simulink subsystem "BatteryHV_SystemTable_refsub"  (R2025b)
settings: Solver=VariableStepAuto  StartTime=0.0  StopTime=10.0  RelTol=1e-3
undefined symbols (not defined in the file or in its folder): batteryHV, initial, Minus, Plus
libraries: fl_lib x24, nesl_utility x10, batteryecm_lib x1
settings Model: Creator=isaacito  LastModifiedBy=isaacito
settings OptimizationCC: ReuseModelBlockBuffer=off
settings RTWCC: GPUComputeCapability=3.5

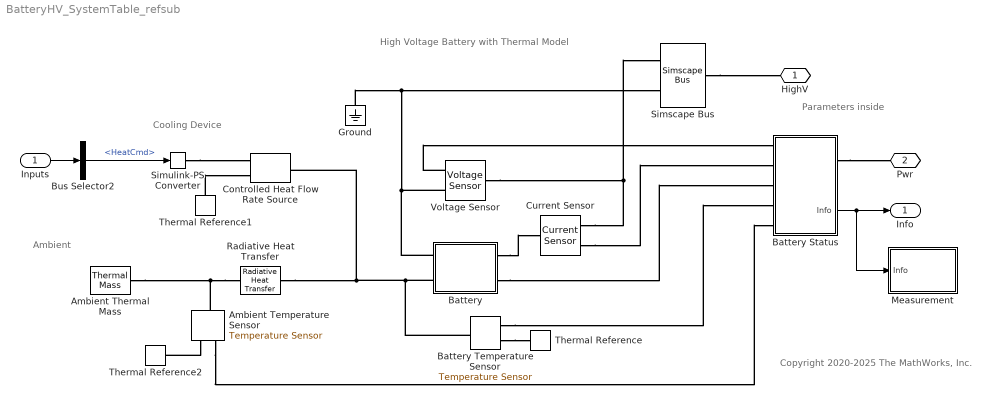
== system BatteryHV_SystemTable_refsub ==
  note: High Voltage Battery with Thermal Model
  note: Ambient
  note: Cooling Device
  note: Copyright 2020-2025 The MathWorks, Inc.
  note: Parameters inside
  Inputs : Inport
  Ambient Temperature Sensor : fl_lib/Thermal/Thermal Sensors/Temperature Sensor  temperature_measure=foundation.enum.MeasurementReference.difference
  Ambient Thermal Mass : fl_lib/Thermal/Thermal Elements/Thermal Mass  mass_type=foundation.enum.constant_variable.constant  mass=batteryHV.ambientMass_t t  sp_heat=batteryHV.ambientSpecificHeat_J_per_Kkg J/(K*kg)  mass_min=1e-6 kg  num_ports=foundation.enum.numPorts2.one  m_specify=off  m_priority=High  m=1 kg  m_nominal_specify=off  m_nominal_value=1  m_nominal_unit=kg  T_specify=on  T_priority=High  T=initial.ambientTemp_K K  T_nominal_specify=off  T_nominal_value=1  T_nominal_unit=K  Q_specify=off  Q_priority=None  Q=0 W  Q_nominal_specify=off  Q_nominal_value=1  Q_nominal_unit=W
  Battery : Subsystem
  Battery Status : Subsystem
      settings: PortSchema="{\"entries\":[{\"content\":{\"sides\":[{\"content\":{\"connectorIds\":[\"LConn1\",\"LConn2\",\"LConn3\",\"LConn4\",\"LConn5\"]},\"type\":\"ConnectorPlacement.EquallySpacedRectSide\",\"uuid\":\"ceb40bee-a67a-415b-b9a3-f68aa0f1718c\"},{\"content\":{\"connectorIds\":[\"RConn1\",\"Out1\"],\"side\":\"RIGHT\"},\"type\":\"ConnectorPlacement.EquallySpacedRectSide\",\"uuid\":\"395c2f85-e3a4-4d83-be11-c4910c287b37\"},{\"content\":{\"side\":\"TOP\"},\"type\":\"ConnectorPlacement.EquallySpacedRectSide\",\"uuid\":\"f70bb581-3c81-49dd-9a63-28b015635667\"}]},\"type\":\"ConnectorPlacement.EquallySpacedConnector\",\"uuid\":\"f11b0a3f-3785-405e-864d-e7b7ac2aade7\"}],\"packageUris\":[\"http://schema.mathworks.com/mf0/Connector/R2020b\"],\"version\":\"1.0\"}"
  Battery Temperature Sensor : fl_lib/Thermal/Thermal Sensors/Temperature Sensor  temperature_measure=foundation.enum.MeasurementReference.difference
  Bus Selector2 : BusSelector  OutputSignals=HeatCmd
  Controlled Heat Flow Rate Source : fl_lib/Thermal/Thermal Sources/Controlled Heat Flow Rate Source
  Current Sensor : fl_lib/Electrical/Electrical Sensors/Current Sensor
  Ground : fl_lib/Electrical/Electrical Elements/Electrical Reference
  Measurement : Subsystem
  Radiative Heat Transfer : fl_lib/Thermal/Thermal Elements/Radiative Heat Transfer  area=batteryHV.RadiationArea_m2 m^2  rad_tr_coeff=batteryHV.RadiationCoeff_W_per_K4m2 W/(K^4*m^2)  T_specify=off  T_priority=None  T=0 K  T_nominal_specify=off  T_nominal_value=1  T_nominal_unit=K  Q_specify=off  Q_priority=None  Q=0 W  Q_nominal_specify=off  Q_nominal_value=1  Q_nominal_unit=W
      settings: InternalSimscapePortConfiguration="{\"Bottom\":[],\"Left\":[{\"id\":\"A\",\"label\":\"A\",\"type\":\"foundation.thermal.thermal\"}],\"Right\":[{\"id\":\"B\",\"label\":\"B\",\"type\":\"foundation.thermal.thermal\"}],\"Top\":[]}"
  Simscape Bus : SimscapeBus  HierarchyStrings=Plus;Minus  ConnectionType=Bus: Bus_HighVoltage
      settings: AttributesFormatString=%<ConnectionType>
  Simulink-PS Converter : nesl_utility/Simulink-PS Converter  PhysicalDomain=network_engine_domain  SubClassName=ps_input  LeftPortType=input  RightPortType=output  PseudoPeriodic=off  Frequencies=[]  NoiseDistribution=none  NoiseParameters=[]  Unit=W  AffineConversion=off  FilteringAndDerivatives=provide  SimscapeFilterOrder=1  InputFilterTimeConstant=0.001  UdotUserProvided=0
  Thermal Reference : fl_lib/Thermal/Thermal Elements/Thermal Reference
  Thermal Reference1 : fl_lib/Thermal/Thermal Elements/Thermal Reference
  Thermal Reference2 : fl_lib/Thermal/Thermal Elements/Thermal Reference
  Voltage Sensor : fl_lib/Electrical/Electrical Sensors/Voltage Sensor
  HighV : PMIOPort  Side=Right
  Pwr : PMIOPort  Port=2  Side=Right
  Info : Outport
  wires:
  Bus Selector2/1 -> Simulink-PS Converter/1  "<HeatCmd>"
  Inputs/1 -> Bus Selector2/1
  Battery Status/1(Info) -> Info/1, Measurement/1(Info)
  connections:
  Ground/LConn1 -- Simscape Bus/LConn2 -- Voltage Sensor/RConn2 -- Battery/RConn1
  Voltage Sensor/LConn1 -- Simscape Bus/LConn1 -- Current Sensor/RConn2
  Battery Temperature Sensor/LConn1 -- Controlled Heat Flow Rate Source/LConn1 -- Radiative Heat Transfer/RConn1 -- Battery/RConn2
  Radiative Heat Transfer/LConn1 -- Ambient Thermal Mass/LConn1 -- Ambient Temperature Sensor/LConn1
  Simscape Bus/RConn1 -- HighV/RConn1
  Ambient Temperature Sensor/RConn1 -- Thermal Reference2/LConn1
  Simulink-PS Converter/RConn1 -- Controlled Heat Flow Rate Source/RConn1
  Thermal Reference1/LConn1 -- Controlled Heat Flow Rate Source/RConn2
  Voltage Sensor/RConn1 -- Battery Status/LConn1
  Current Sensor/RConn1 -- Battery Status/LConn2
  Battery Temperature Sensor/RConn1 -- Thermal Reference/LConn1
  Battery Temperature Sensor/RConn2 -- Battery Status/LConn4
  Ambient Temperature Sensor/RConn2 -- Battery Status/LConn5
  Battery/LConn2 -- Battery Status/LConn3
  Battery/LConn1 -- Current Sensor/LConn1
  Battery Status/RConn1 -- Pwr/RConn1

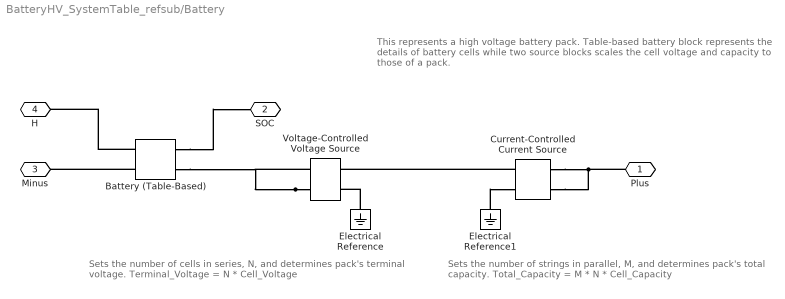
== system BatteryHV_SystemTable_refsub/Battery ==
  note: This represents a high voltage battery pack.
      | Table-based battery block represents the details of
      | battery cells while two source blocks scales
      | the cell voltage and capacity to those of a pack.
  note: Sets the number of strings in parallel, M,
      | and determines pack's total capacity.
      | Total_Capacity = M * N * Cell_Capacity
  note: Sets the number of cells in series, N,
      | and determines pack's terminal voltage.
      | Terminal_Voltage = N * Cell_Voltage
  Battery (Table-Based) : batteryecm_lib/Battery (Table-Based)  SOC_vec=batteryHV.SOC_normalized  T_dependence=simscape.enum.tablebattery.temperature_dependence.yes  prm_dir=simscape.enum.tablebattery.prm_dir.noCurrentDirectionality  T_vec=batteryHV.Temperatures_degC degC  V0_mat=batteryHV.OpenCircuitVoltage_V V  V0_vec=[3.5057, 3.566, 3.6337, 3.7127, 3.9259, 4.0777, 4.1928] V  V_range=[0, inf] V  R0_mat=batteryHV.TerminalResistance_Ohm Ohm  R0_vec=[.0085, .0085, .0087, .0082, .0083, .0085, .0085] Ohm  R0_dis_mat=[.0117, .0085, .009; .011, .0085, .009; .0114, .0087, .0092; .0107, .0082, .0088; .0107, .0083, .0091; .0113, .0085, .0089; .0116, .0085, .0089] Ohm  R0_dis_vec=[.0085, .0085, .0087, .0082, .0083, .0085, .0085] Ohm  R0_ch_mat=[.0117, .0085, .009; .011, .0085, .009; .0114, .0087, .0092; .0107, .0082, .0088; .0107, .0083, .0091; .0113, .0085, .0089; .0116, .0085, .0089] Ohm  R0_ch_vec=[.0085, .0085, .0087, .0082, .0083, .0085, .0085] Ohm  AH=batteryHV.CellCharge_Ahr A*hr  prm_leak=simscape.enum.tablebattery.prm_leak.disabled  Rleak_vec=[8000, 7000, 6000] Ohm  Rleak=7e3 Ohm  extrapolation_option=simscape.enum.extrapolation.nearest  SOC_port=simscape.enum.tablebattery.enable.yes  prm_dyn=simscape.enum.tablebattery.prm_dyn.off  R1_mat=[.0109, .0029, .0013; .0069, .0024, .0012; .0047, .0026, .0013; .0034, .0016, .001; .0033, .0023, .0014; .0033, .0018, .0011; .0028, .0017, .0011] Ohm  R1_vec=[.0029, .0024, .0026, .0016, .0023, .0018, .0017] Ohm  tau1_mat=[20, 36, 39; 31, 45, 39; 109, 105, 61; 36, 29, 26; 59, 77, 67; 40, 33, 29; 25, 39, 33] s  tau1_vec=[36, 45, 105, 29, 77, 33, 39] s  R2_mat=[.0109, .0029, .0013; .0069, .0024, .0012; .0047, .0026, .0013; .0034, .0016, .001; .0033, .0023, .0014; .0033, .0018, .0011; .0028, .0017, .0011] Ohm  R2_vec=[.0029, .0024, .0026, .0016, .0023, .0018, .0017] Ohm  tau2_mat=[20, 36, 39; 31, 45, 39; 109, 105, 61; 36, 29, 26; 59, 77, 67; 40, 33, 29; 25, 39, 33] s  tau2_vec=[36, 45, 105, 29, 77, 33, 39] s  R3_mat=[.0109, .0029, .0013; .0069, .0024, .0012; .0047, .0026, .0013; .0034, .0016, .001; .0033, .0023, .0014; .0033, .0018, .0011; .0028, .0017, .0011] Ohm  R3_vec=[.0029, .0024, .0026, .0016, .0023, .0018, .0017] Ohm  tau3_mat=[20, 36, 39; 31, 45, 39; 109, 105, 61; 36, 29, 26; 59, 77, 67; 40, 33, 29; 25, 39, 33] s  tau3_vec=[36, 45, 105, 29, 77, 33, 39] s  R4_mat=[.0109, .0029, .0013; .0069, .0024, .0012; .0047, .0026, .0013; .0034, .0016, .001; .0033, .0023, .0014; .0033, .0018, .0011; .0028, .0017, .0011] Ohm  R4_vec=[.0029, .0024, .0026, .0016, .0023, .0018, .0017] Ohm  tau4_mat=[20, 36, 39; 31, 45, 39; 109, 105, 61; 36, 29, 26; 59, 77, 67; 40, 33, 29; 25, 39, 33] s  tau4_vec=[36, 45, 105, 29, 77, 33, 39] s  R5_mat=[.0109, .0029, .0013; .0069, .0024, .0012; .0047, .0026, .0013; .0034, .0016, .001; .0033, .0023, .0014; .0033, .0018, .0011; .0028, .0017, .0011] Ohm  R5_vec=[.0029, .0024, .0026, .0016, .0023, .0018, .0017] Ohm  tau5_mat=[20, 36, 39; 31, 45, 39; 109, 105, 61; 36, 29, 26; 59, 77, 67; 40, 33, 29; 25, 39, 33] s  tau5_vec=[36, 45, 105, 29, 77, 33, 39] s  prm_fade=simscape.enum.tablebattery.prm_fade.disabled  N0=100  dV0=0  dR0=0  dAH=0  dRleak=0  dR1=0  dR2=0  dR3=0  dR4=0  dR5=0  N0vec=[100, 200, 300]  Tfadevec=[298.15, 323.15] K  dV0vec=[0, 0, 0]  dR0vec=[0, 0, 0]  dAHvec=[0, 0, 0]  dRleakvec=[0, 0, 0]  dR1vec=[0, 0, 0]  dR2vec=[0, 0, 0]  dR3vec=[0, 0, 0]  dR4vec=[0, 0, 0]  dR5vec=[0, 0, 0]  dV0mat=[0, 0; 0, 0; 0, 0]  dR0mat=[0, 0; 0, 0; 0, 0]  dAHmat=[0, 0; 0, 0; 0, 0]  dRleakmat=[0, 0; 0, 0; 0, 0]  dR1mat=[0, 0; 0, 0; 0, 0]  dR2mat=[0, 0; 0, 0; 0, 0]  dR3mat=[0, 0; 0, 0; 0, 0]  dR4mat=[0, 0; 0, 0; 0, 0]  dR5mat=[0, 0; 0, 0; 0, 0]  prm_age_modeling=simscape.enum.tablebattery.prm_age_modeling.equation  storage_dt_age_vec=[0] d  storage_T_age_vec=[273] K  prm_age_OCV=simscape.enum.tablebattery.prm_age_OCV.OCV  OCV_age=0.9  SOC_age=0.6  prm_age_resistance=simscape.enum.tablebattery.prm_age.disabled  OCV_scaling_age_resistance=2.2134e6  OCV_offset_age_resistance=1.632e6  temp_exp_age_resistance=0.515833569 V  t_exp_age_resistance=0.75  T_age_vec_resistance=[273.15, 298.15, 323.15] K  dt_age_vec_resistance=[90, 180, 270, 360] d  dR0_age_vec=[0, 0, 0]  t_meas_dR0_age=100 d  dR0_age_mat=[0, 0, 0; 0, 0, 0; 0, 0, 0; 0, 0, 0]  prm_age_capacity=simscape.enum.tablebattery.prm_age.disabled  OCV_scaling_age_capacity=1.5097e07  OCV_offset_age_capacity=8.3625e06  temp_exp_age_capacity=0.6011 V  t_exp_age_capacity=0.75  T_age_vec_capacity=[273.15, 298.15, 323.15] K  dt_age_vec_capacity=[90, 180, 270, 360] d  dAH_age_vec=[0, 0, 0]  t_meas_dAH_age=100 d  dAH_age_mat=[0, 0, 0; 0, 0, 0; 0, 0, 0; 0, 0, 0]  thermal_port=simscape.enum.thermaleffects.model  temperature=298.15 K  thermal_mass=batteryHV.ThermalMassOfAllCells_J_per_K J/K  i_specify=off  i_priority=None  i=0 A  i_nominal_specify=off  i_nominal_value=1  i_nominal_unit=A  v_specify=off  v_priority=None  v=0 V  v_nominal_specify=off  v_nominal_value=1  v_nominal_unit=V  stateOfCharge_specify=on  stateOfCharge_priority=High  stateOfCharge=initial.hvBattery_SOC_normalized  stateOfCharge_nominal_specify=off  stateOfCharge_nominal_value=1  stateOfCharge_nominal_unit=1  num_cycles_specify=off  num_cycles_priority=High  num_cycles=0  num_cycles_nominal_specify=off  num_cycles_nominal_value=1  num_cycles_nominal_unit=1  cell_temperature_specify=on  cell_temperature_priority=High  cell_temperature=initial.hvBattery_Temperature_K K  cell_temperature_nominal_specify=off  cell_temperature_nominal_value=1  cell_temperature_nominal_unit=K
  Current-Controlled Current Source : fl_lib/Electrical/Electrical Sources/Current-Controlled Current Source  K=batteryHV.CurrentGain  i1_specify=off  i1_priority=None  i1=0 A  i1_nominal_specify=off  i1_nominal_value=1  i1_nominal_unit=A  i2_specify=off  i2_priority=None  i2=0 A  i2_nominal_specify=off  i2_nominal_value=1  i2_nominal_unit=A
      settings: InternalSimscapePortConfiguration="{\"Bottom\":[],\"Left\":[{\"id\":\"p1\",\"label\":\"+\",\"type\":\"foundation.electrical.electrical\"},{\"id\":\"head\",\"label\":\"\",\"type\":\"foundation.electrical.electrical\"}],\"Right\":[{\"id\":\"n1\",\"label\":\"-\",\"type\":\"foundation.electrical.electrical\"},{\"id\":\"tail\",\"label\":\"\",\"type\":\"foundation.electrical.electrical\"}],\"Top\":[]}"
  Electrical Reference : fl_lib/Electrical/Electrical Elements/Electrical Reference
  Electrical Reference1 : fl_lib/Electrical/Electrical Elements/Electrical Reference
  Voltage-Controlled Voltage Source : fl_lib/Electrical/Electrical Sources/Voltage-Controlled Voltage Source  K=batteryHV.VoltageGain  v1_specify=off  v1_priority=None  v1=0 V  v1_nominal_specify=off  v1_nominal_value=1  v1_nominal_unit=V  v2_specify=off  v2_priority=None  v2=0 V  v2_nominal_specify=off  v2_nominal_value=1  v2_nominal_unit=V
      settings: InternalSimscapePortConfiguration="{\"Bottom\":[],\"Left\":[{\"id\":\"p1\",\"label\":\"+\",\"type\":\"foundation.electrical.electrical\"},{\"id\":\"p2\",\"label\":\"+\",\"type\":\"foundation.electrical.electrical\"}],\"Right\":[{\"id\":\"n1\",\"label\":\"-\",\"type\":\"foundation.electrical.electrical\"},{\"id\":\"n2\",\"label\":\"-\",\"type\":\"foundation.electrical.electrical\"}],\"Top\":[]}"
  Plus : PMIOPort  Side=Left
  SOC : PMIOPort  Port=2  Side=Left
  Minus : PMIOPort  Port=3  Side=Right
  H : PMIOPort  Port=4  Side=Right
  connections:
  Electrical Reference1/LConn1 -- Current-Controlled Current Source/LConn2
  Electrical Reference/LConn1 -- Voltage-Controlled Voltage Source/LConn1
  Voltage-Controlled Voltage Source/RConn1 -- Voltage-Controlled Voltage Source/RConn2 -- Battery (Table-Based)/LConn1
  Current-Controlled Current Source/LConn1 -- Voltage-Controlled Voltage Source/LConn2
  Plus/RConn1 -- Current-Controlled Current Source/RConn1 -- Current-Controlled Current Source/RConn2
  Battery (Table-Based)/RConn1 -- Minus/RConn1
  Battery (Table-Based)/LConn2 -- SOC/RConn1
  Battery (Table-Based)/RConn2 -- H/RConn1

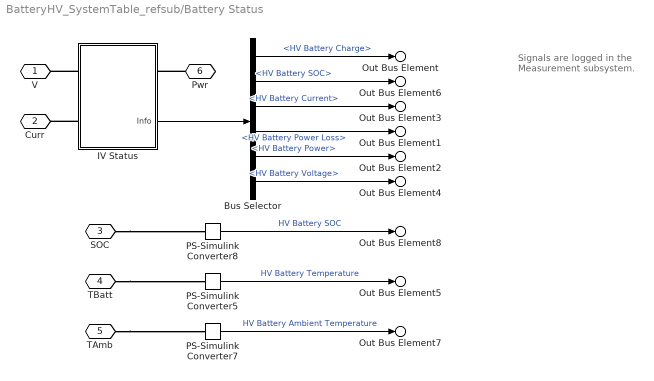
== system BatteryHV_SystemTable_refsub/Battery Status ==
  note: Signals are logged in
      | the Measurement subsystem.
  Bus Selector : BusSelector  OutputSignals=HV Battery Charge,HV Battery SOC,HV Battery Current,HV Battery Power Loss,HV Battery Power,HV Battery Voltage
  IV Status : Subsystem
      settings: PortSchema="{\"entries\":[{\"content\":{\"sides\":[{\"content\":{\"connectorIds\":[\"LConn1\",\"LConn2\"]},\"type\":\"ConnectorPlacement.EquallySpacedRectSide\",\"uuid\":\"fa3fe2c3-d9c0-40ca-976a-fdfa614694fc\"},{\"content\":{\"connectorIds\":[\"RConn1\",\"Out1\"],\"side\":\"RIGHT\"},\"type\":\"ConnectorPlacement.EquallySpacedRectSide\",\"uuid\":\"d6ed96ef-770b-4a18-8b31-ef7e8f253069\"},{\"content\":{\"side\":\"TOP\"},\"type\":\"ConnectorPlacement.EquallySpacedRectSide\",\"uuid\":\"d9a8161e-0196-4518-8226-4ae50c8bd457\"}]},\"type\":\"ConnectorPlacement.EquallySpacedConnector\",\"uuid\":\"0aac0953-a631-4fd0-93f3-a84e629f2b58\"}],\"packageUris\":[\"http://schema.mathworks.com/mf0/Connector/R2020b\"],\"version\":\"1.0\"}"
  PS-Simulink Converter5 : nesl_utility/PS-Simulink Converter  PhysicalDomain=network_engine_domain  SubClassName=ps_output  LeftPortType=input  RightPortType=output  PseudoPeriodic=off  Frequencies=[]  VectorFormat=inherit  Unit=degC  AffineConversion=on
  PS-Simulink Converter7 : nesl_utility/PS-Simulink Converter  PhysicalDomain=network_engine_domain  SubClassName=ps_output  LeftPortType=input  RightPortType=output  PseudoPeriodic=off  Frequencies=[]  VectorFormat=inherit  Unit=degC  AffineConversion=on
  PS-Simulink Converter8 : nesl_utility/PS-Simulink Converter  PhysicalDomain=network_engine_domain  SubClassName=ps_output  LeftPortType=input  RightPortType=output  PseudoPeriodic=off  Frequencies=[]  VectorFormat=1-D array  Unit=1  AffineConversion=off
  V : PMIOPort  Side=Left
  Curr : PMIOPort  Port=2  Side=Left
  SOC : PMIOPort  Port=3  Side=Left
  TBatt : PMIOPort  Port=4  Side=Left
  TAmb : PMIOPort  Port=5  Side=Left
  Pwr : PMIOPort  Port=6  Side=Right
  Out Bus Element5 : Outport  PortName=Info  Element=Temp
      settings: AttributesFormatString=%<Unit>
  Out Bus Element7 : Outport  PortName=Info  Element=TempAmb
      settings: AttributesFormatString=%<Unit>
  Out Bus Element8 : Outport  PortName=Info  Element=trueSOC
      settings: AttributesFormatString=%<Unit>
  Out Bus Element : Outport  PortName=Info  Element=Charge
  Out Bus Element3 : Outport  PortName=Info  Element=Current
  Out Bus Element1 : Outport  PortName=Info  Element=PowerLoss
  Out Bus Element2 : Outport  PortName=Info  Element=Power
  Out Bus Element4 : Outport  PortName=Info  Element=Voltage
  Out Bus Element6 : Outport  PortName=Info  Element=SOC
  wires:
  PS-Simulink Converter7/1 -> Out Bus Element7/1  "HV Battery Ambient Temperature"
  PS-Simulink Converter5/1 -> Out Bus Element5/1  "HV Battery Temperature"
  PS-Simulink Converter8/1 -> Out Bus Element8/1  "HV Battery SOC"
  Bus Selector/2 -> Out Bus Element6/1  "<HV Battery SOC>"
  Bus Selector/4 -> Out Bus Element1/1  "<HV Battery Power Loss>"
  Bus Selector/1 -> Out Bus Element/1  "<HV Battery Charge>"
  Bus Selector/5 -> Out Bus Element2/1  "<HV Battery Power>"
  Bus Selector/6 -> Out Bus Element4/1  "<HV Battery Voltage>"
  IV Status/1(Info) -> Bus Selector/1
  Bus Selector/3 -> Out Bus Element3/1  "<HV Battery Current>"
  connections:
  TAmb/RConn1 -- PS-Simulink Converter7/LConn1
  TBatt/RConn1 -- PS-Simulink Converter5/LConn1
  SOC/RConn1 -- PS-Simulink Converter8/LConn1
  IV Status/LConn2 -- Curr/RConn1
  IV Status/LConn1 -- V/RConn1
  Pwr/RConn1 -- IV Status/RConn1

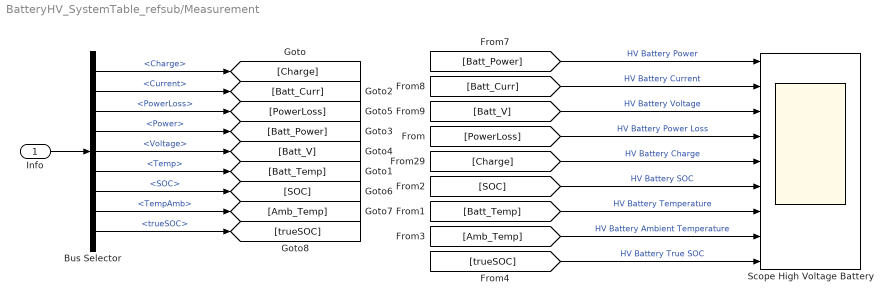
== system BatteryHV_SystemTable_refsub/Measurement ==
  Info : Inport
  Bus Selector : BusSelector  OutputSignals=Charge,Current,PowerLoss,Power,Voltage,Temp,SOC,TempAmb,trueSOC
  Scope High Voltage Battery : Scope  NumInputPorts=9
      settings: ActiveDisplayYMinimum=-2.22148  ActiveDisplayYMaximum=4.24683
  wires:
  [trueSOC] -> Scope High Voltage Battery/9  "HV Battery True SOC"
  Bus Selector/9 -> [trueSOC]  "<trueSOC>"
  [SOC] -> Scope High Voltage Battery/6  "HV Battery SOC"
  [Amb_Temp] -> Scope High Voltage Battery/8  "HV Battery Ambient Temperature"
  [Batt_Temp] -> Scope High Voltage Battery/7  "HV Battery Temperature"
  Bus Selector/7 -> [SOC]  "<SOC>"
  [Charge] -> Scope High Voltage Battery/5  "HV Battery Charge"
  [PowerLoss] -> Scope High Voltage Battery/4  "HV Battery Power Loss"
  Bus Selector/2 -> [Batt_Curr]  "<Current>"
  Bus Selector/4 -> [Batt_Power]  "<Power>"
  [Batt_V] -> Scope High Voltage Battery/3  "HV Battery Voltage"
  Bus Selector/6 -> [Batt_Temp]  "<Temp>"
  [Batt_Power] -> Scope High Voltage Battery/1  "HV Battery Power"
  Bus Selector/8 -> [Amb_Temp]  "<TempAmb>"
  [Batt_Curr] -> Scope High Voltage Battery/2  "HV Battery Current"
  Bus Selector/5 -> [Batt_V]  "<Voltage>"
  Info/1 -> Bus Selector/1
  Bus Selector/3 -> [PowerLoss]  "<PowerLoss>"
  Bus Selector/1 -> [Charge]  "<Charge>"

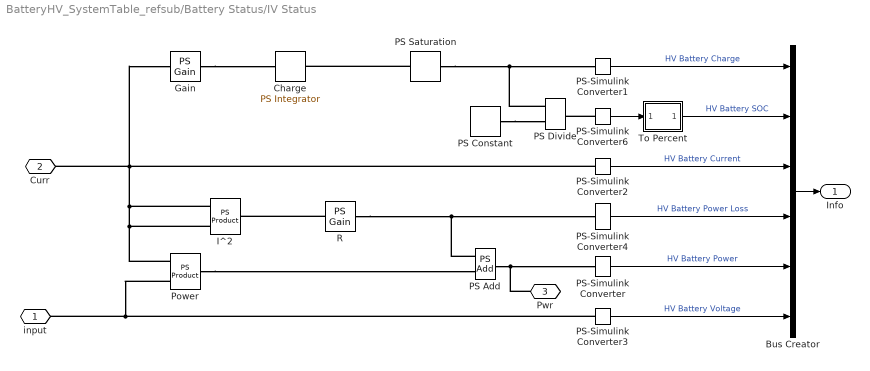
== system BatteryHV_SystemTable_refsub/Battery Status/IV Status ==
  Bus Creator : BusCreator  Inputs=6
  Charge : fl_lib/Physical Signals/Linear Operators/PS Integrator  reset_method=foundation.enum.IntegratorResetSpec.None  initial_condition_spec=foundation.enum.IntegratorICSpec.Internal  saturation_spec=foundation.enum.IntegratorSaturationSpec.None  saturation_source_spec=foundation.enum.IntegratorSaturationSourceSpec.Internal  x0=initial.hvBattery_Charge_Ahr A*hr  xu=inf s  xl=-inf s
      settings: AttributesFormatString=%<x0> [%<x0_unit>]
  Gain : fl_lib/Physical Signals/Functions/PS Gain  gain=-1
      settings: AttributesFormatString=%<gain>
  I^2 : fl_lib/Physical Signals/Functions/PS Product
  PS Add : fl_lib/Physical Signals/Functions/PS Add
  PS Constant : fl_lib/Physical Signals/Sources/PS Constant  constant=batteryHV.nominalCharge_Ahr A*hr
      settings: AttributesFormatString=%<constant> [%<constant_unit>]
  PS Divide : fl_lib/Physical Signals/Functions/PS Divide
  PS Saturation : fl_lib/Physical Signals/Nonlinear Operators/PS Saturation  upper_limit=batteryHV.nominalCharge_Ahr A*hr  lower_limit=0 A*hr  ZeroCross=true
      settings: AttributesFormatString=|
      | Upper: %<upper_limit>
      | Lower: %<lower_limit>
  PS-Simulink Converter : nesl_utility/PS-Simulink Converter  PhysicalDomain=network_engine_domain  SubClassName=ps_output  LeftPortType=input  RightPortType=output  PseudoPeriodic=off  Frequencies=[]  VectorFormat=1-D array  Unit=kW  AffineConversion=off
  PS-Simulink Converter1 : nesl_utility/PS-Simulink Converter  PhysicalDomain=network_engine_domain  SubClassName=ps_output  LeftPortType=input  RightPortType=output  PseudoPeriodic=off  Frequencies=[]  VectorFormat=1-D array  Unit=A*hr  AffineConversion=off
  PS-Simulink Converter2 : nesl_utility/PS-Simulink Converter  PhysicalDomain=network_engine_domain  SubClassName=ps_output  LeftPortType=input  RightPortType=output  PseudoPeriodic=off  Frequencies=[]  VectorFormat=1-D array  Unit=A  AffineConversion=off
  PS-Simulink Converter3 : nesl_utility/PS-Simulink Converter  PhysicalDomain=network_engine_domain  SubClassName=ps_output  LeftPortType=input  RightPortType=output  PseudoPeriodic=off  Frequencies=[]  VectorFormat=1-D array  Unit=V  AffineConversion=off
  PS-Simulink Converter4 : nesl_utility/PS-Simulink Converter  PhysicalDomain=network_engine_domain  SubClassName=ps_output  LeftPortType=input  RightPortType=output  PseudoPeriodic=off  Frequencies=[]  VectorFormat=1-D array  Unit=W  AffineConversion=off
  PS-Simulink Converter6 : nesl_utility/PS-Simulink Converter  PhysicalDomain=network_engine_domain  SubClassName=ps_output  LeftPortType=input  RightPortType=output  PseudoPeriodic=off  Frequencies=[]  VectorFormat=inherit  Unit=1  AffineConversion=off
  Power : fl_lib/Physical Signals/Functions/PS Product
  R : fl_lib/Physical Signals/Functions/PS Gain  gain=batteryHV.internalResistance_Ohm Ohm
      settings: AttributesFormatString=%<gain> [%<gain_unit>]
  To Percent : Subsystem
  input : PMIOPort  Side=Left
  Curr : PMIOPort  Port=2  Side=Left
  Pwr : PMIOPort  Port=3  Side=Right
  Info : Outport
  wires:
  To Percent/1(Out1) -> Bus Creator/2  "HV Battery SOC"
  PS-Simulink Converter4/1 -> Bus Creator/4  "HV Battery Power Loss"
  PS-Simulink Converter3/1 -> Bus Creator/6  "HV Battery Voltage"
  PS-Simulink Converter1/1 -> Bus Creator/1  "HV Battery Charge"
  PS-Simulink Converter6/1 -> To Percent/1(In1)
  PS-Simulink Converter2/1 -> Bus Creator/3  "HV Battery Current"
  PS-Simulink Converter/1 -> Bus Creator/5  "HV Battery Power"
  Bus Creator/1 -> Info/1
  connections:
  PS Add/RConn1 -- Pwr/RConn1 -- PS-Simulink Converter/LConn1
  Power/RConn1 -- PS Add/LConn2
  PS Saturation/LConn1 -- Charge/RConn1
  PS Divide/LConn1 -- PS-Simulink Converter1/LConn1 -- PS Saturation/RConn1
  Power/LConn2 -- I^2/LConn1 -- I^2/LConn2 -- PS-Simulink Converter2/LConn1 -- Gain/LConn1 -- Curr/RConn1
  Power/LConn1 -- PS-Simulink Converter3/LConn1 -- input/RConn1
  PS Constant/RConn1 -- PS Divide/LConn2
  Gain/RConn1 -- Charge/LConn1
  PS-Simulink Converter6/LConn1 -- PS Divide/RConn1
  R/LConn1 -- I^2/RConn1
  R/RConn1 -- PS-Simulink Converter4/LConn1 -- PS Add/LConn1

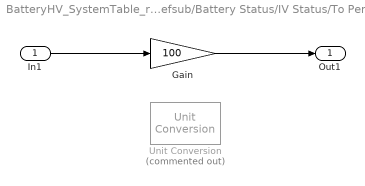
== system BatteryHV_SystemTable_refsub/Battery Status/IV Status/To Percent ==
  In1 : Inport
  Gain : Gain  Gain=100
  Unit Conversion : UnitConversion  Commented=on
  Out1 : Outport  Unit=%
      settings: AttributesFormatString=%<Unit>
  wires:
  In1/1 -> Gain/1
  Gain/1 -> Out1/1
